simulink model "appendix02_Bicopter_ClosedLoop_PID"  (R2026b)
settings: Solver=FixedStepAuto  StopTime=inf  EnableMultiTasking=on
undefined symbols (not defined in the file or in its folder): ODR
libraries: arduinolib x6, arduinowifilib x2, arduinosensorlib x1, slpidlib x1
settings Model: SILPILModeSetting=veronly  Creator=lcree  LastModifiedBy=ayeo
settings OptimizationCC: DifferentSizesBufferReuse=on  EnhancedBackFolding=on  MaxStackSize=64  OptimizationCustomize=off  OptimizeBlockOrder=speed
settings DebuggingCC: ParameterPrecisionLossMsg=none  ParameterTunabilityLossMsg=error
settings HardwareCC: ProdHWDeviceType=ARM Compatible->ARM Cortex  ProdLargestAtomicFloat=Double  ProdLargestAtomicInteger=Long  UseEmbeddedCoderFeatures=off  UseSimulinkCoderFeatures=off
settings SFSimCC: MATLABDynamicMemAlloc=off
settings RTWCC: BuildConfiguration=Faster Runs  Description=Embedded Coder  HardwareBoard=Arduino Nano 33 IoT  SystemTargetFile=ert.tlc  TLCOptions=-aInlineSetEventsForThisBaseRateFcn=TLC_FALSE -aSuppressMultiTaskScheduler=TLC_FALSE -aRateBasedStepFcn=1  TemplateMakefile=ert_default_tmf  Toolchain=Arduino ARM
settings CodeAppCC: ForceParamTrailComments=on  OperatorAnnotations=on
settings ERTTargetCC: DynamicArrayContainerType=coder::array  ERTCustomFileBanners=off  ExtModeIntrfLevel=Level2 - Open  ExtModeMexFile=ext_xcp  ExtModeStaticAlloc=on  ModelStepFunctionPrototypeControlCompliant=off  SupportContinuousTime=on  SupportNonInlinedSFcns=on  SupportVariableSizeSignals=on

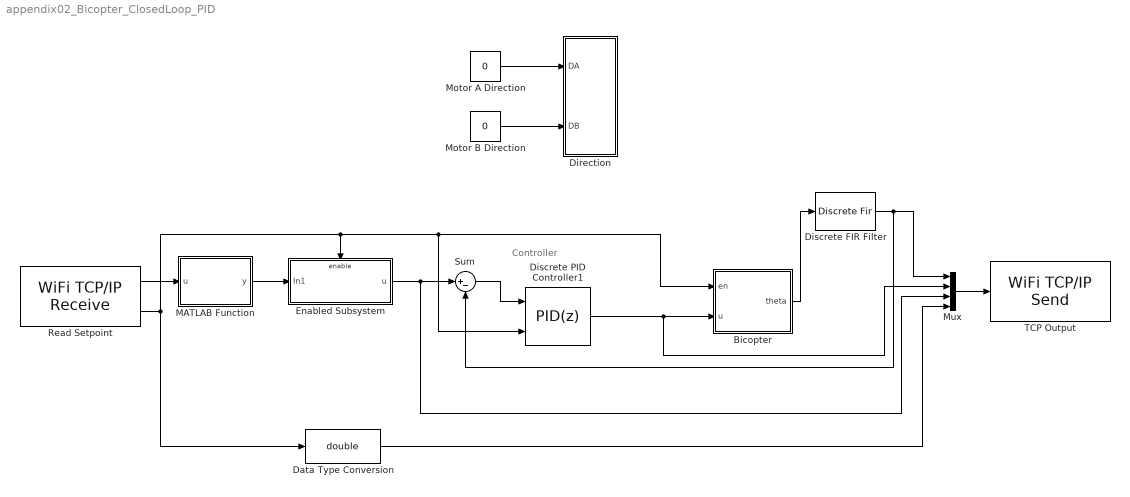
== system appendix02_Bicopter_ClosedLoop_PID ==
  note: Controller
  Bicopter : Subsystem
  Data Type Conversion : DataTypeConversion  OutDataTypeStr=double  SaturateOnIntegerOverflow=off  RndMeth=Floor
  Direction : Subsystem
  Discrete FIR Filter : DiscreteFir  Coefficients=0.1*ones(1,10)  OutDataTypeStr=Inherit: Same as accumulator
  Discrete PID Controller1 : slpidlib/PID Controller  Controller=PID  Form=Parallel  TimeDomain=Discrete-time  UseExternalTs=off  SampleTime=0.01  IntegratorMethod=Backward Euler  FilterMethod=Backward Euler  ControllerParametersSource=internal  P=15.49  I=33.59  UseKiTs=off  D=0  UseExternalDerivativeSource=off  N=100  UseFilter=on  TunerSelectOption=Frequency Response Based  InitialConditionSource=internal  InitialConditionForIntegrator=0  InitialConditionForFilter=0  DifferentiatorICPrevScaledInput=-10  ExternalReset=rising  TrackingMode=off  Kt=1  LimitOutput=off  SatLimitsSource=internal  UpperSaturationLimit=inf  LowerSaturationLimit=-inf  LinearizeAsGain=off  AntiWindupMode=none  Kb=1  LimitIntegrator=off  UpperIntegratorSaturationLimit=inf  LowerIntegratorSaturationLimit=-inf  POutMin=[]  POutMax=[]  IOutMin=[]  IOutMax=[]  DOutMin=[]  DOutMax=[]  NOutMin=[]  NOutMax=[]  SumOutMin=[]  SumOutMax=[]  SaturationOutMin=[]  SaturationOutMax=[]  PParamMin=[]  PParamMax=[]  IParamMin=[]  IParamMax=[]  DParamMin=[]  DParamMax=[]  NParamMin=[]  NParamMax=[]  KbParamMin=[]  KbParamMax=[]  KtParamMin=[]  KtParamMax=[]  KbOutMin=[]  KbOutMax=[]  KtOutMin=[]  KtOutMax=[]  IntegratorOutMin=[]  IntegratorOutMax=[]  FilterOutMin=[]  FilterOutMax=[]  SumI1OutMin=[]  SumI1OutMax=[]  SumI2OutMin=[]  SumI2OutMax=[]  SumI3OutMin=[]  SumI3OutMax=[]  SumI4OutMin=[]  SumI4OutMax=[]  SumDOutMin=[]  SumDOutMax=[]  DifferentiatorOutMin=[]  DifferentiatorOutMax=[]  FilterDiffOutCoefMin=[]  FilterDiffOutCoefMax=[]  ReciprocalOutMin=[]  ReciprocalOutMax=[]  SumDenOutMin=[]  SumDenOutMax=[]  SumNumOutMin=[]  SumNumOutMax=[]  DivideOutMin=[]  DivideOutMax=[]  UdiffTsProdOutMin=[]  UdiffTsProdOutMax=[]  NTsProdOutMin=[]  NTsProdOutMax=[]  UintegralTsProdOutMin=[]  UintegralTsProdOutMax=[]  UngainTsProdOutMin=[]  UngainTsProdOutMax=[]  ClampingZeroOutDataTypeStr=Inherit: Inherit via back propagation  ClampingZeroOutMin=[]  ClampingZeroOutMax=[]  FilterDenConstantOutDataTypeStr=Inherit: Inherit via back propagation  FilterDenConstantOutMin=[]  FilterDenConstantOutMax=[]  PCopyOutDataTypeStr=Inherit: Inherit via back propagation  PCopyOutMin=[]  PCopyOutMax=[]  NCopyOutDataTypeStr=Inherit: Inherit via back propagation  NCopyOutMin=[]  NCopyOutMax=[]  IntegratorContinuousStateAttributes=''  IntegratorStateMustResolveToSignalObject=off  IntegratorRTWStateStorageClass=Auto  FilterContinuousStateAttributes=''  FilterStateMustResolveToSignalObject=off  FilterRTWStateStorageClass=Auto  ParallelPVariant=InternalParameters  IdealPVariant=Disabled  IVariant=InternalParameters  DVariant=InternalParameters  IntegratorVariant=Discrete  SatVariant=Disabled  AWVariant=Passthrough  PCopyVariant=Disabled  TRVariant=Disabled  FdbkBlocksVariant=Forward  IdealPFdbkVariant=Disabled  SatFdbkVariant=Disabled  DerivativeFilterVariant=BackwardEulerFilter  NVariant=InternalParameters  NCopyVariant=InternalParameters  FilterICVariant=InternalICsFilter  IntegratorICVariant=InternalICs  ExternalResetVariant=ExternalReset  TRSumVariant=Passthrough  SumFdbkVariant=Disabled  SumVariant=Sum_PID  TsampFilterVariant=InternalTs  TsampNgainVariant=Passthrough  TsampIntegralVariant=Disabled_SignalSpec  ExternalSaturationOutDataTypeStr=Inherit: Same as second input  DerivativeSourceVariant=ErrorSignal  PreIntVariant=InternalPreInt
  Enabled Subsystem : Subsystem  TreatAsAtomicUnit=on
  MATLAB Function : MATLAB Function  TreatAsAtomicUnit=on
  Motor A Direction : Constant  Value=0  OutDataTypeStr=boolean
  Motor B Direction : Constant  Value=0  OutDataTypeStr=boolean
  Mux : Mux
  Read Setpoint : arduinowifilib/WiFi TCP//IP Receive  Mode_=Server  serverport=25000  RemoteAddr_=192.168.1.2  RemoteServerPort_=25000  DataType_=uint8  DataSize_=4  SampleTime_=0.01  remoteipoctet1=192  remoteipoctet2=168  remoteipoctet3=1  remoteipoctet4=2  wifiTCPServerIndex=0  wifiTCPClientIndex=0  blockPlatform=ARDUINO  isARMArch=true  BlockingMode_=off  BlockTimeout_=1
  Sum : Sum  Inputs=|+-
  TCP Output : arduinowifilib/WiFi TCP//IP Send  Mode_=Server  serverport=25000  RemoteAddr_=192.168.1.2  RemoteServerPort_=25000  remoteipoctet1=192  remoteipoctet2=168  remoteipoctet3=1  remoteipoctet4=2  wifiTCPServerIndex=0  wifiTCPClientIndex=0  blockPlatform=ARDUINO  isARMArch=true
  wires:
  Motor A Direction/1 -> Direction/1(DA)
  Motor B Direction/1 -> Direction/2(DB)
  Mux/1 -> TCP Output/1
  Enabled Subsystem/1(u) -> Sum/1, Mux/3
  Read Setpoint/2 -> Bicopter/1(en), Discrete PID Controller1/2, Enabled Subsystem/Enable, Data Type Conversion/1
  Discrete PID Controller1/1 -> Mux/2, Bicopter/2(u)
  Data Type Conversion/1 -> Mux/4
  Read Setpoint/1 -> MATLAB Function/1(u)
  MATLAB Function/1(y) -> Enabled Subsystem/1(In1)
  Bicopter/1(theta) -> Discrete FIR Filter/1
  Discrete FIR Filter/1 -> Sum/2, Mux/1
  Sum/1 -> Discrete PID Controller1/1

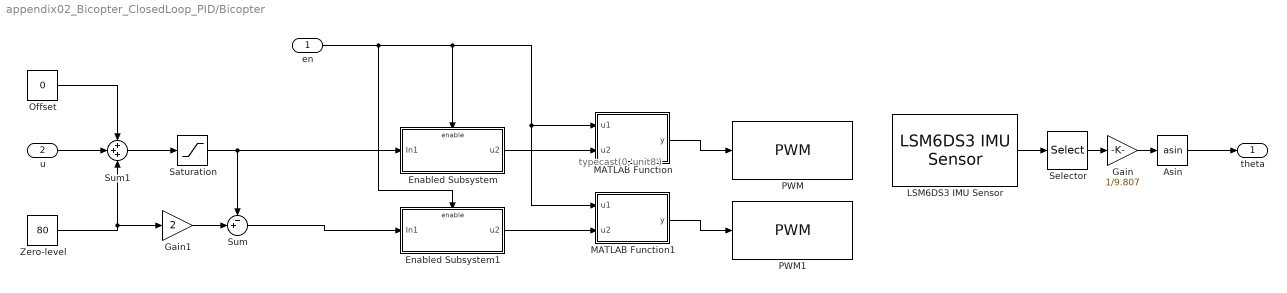
== system appendix02_Bicopter_ClosedLoop_PID/Bicopter ==
  note: typecast(0,'unit8')
  en : Inport
  u : Inport  Port=2
  Asin : Trigonometry  Operator=asin
  Enabled Subsystem : Subsystem  TreatAsAtomicUnit=on
  Enabled Subsystem1 : Subsystem  TreatAsAtomicUnit=on
  Gain : Gain  Gain=1/9.807
  Gain1 : Gain  Gain=2
  LSM6DS3 IMU Sensor : arduinosensorlib/LSM6DS3 IMU Sensor  I2CModule=0  I2CAddress=0x6A  IsActiveAcceleration=on  IsActiveAngularRate=off  IsActiveTemperature=off  IsActiveStatus=off  IsActiveTimeStamp=off  spf=1  SampleTime=0.01  QueueSizeFactor=1  AccelerometerRange=+/- 2g  AccelerometerODR=208 Hz  SelectAnalogBW=off  AccelLPF1BW=400 Hz  AccelSelectCompositeFilter=Low pass filter  AccelLPF2BW=ODR/400  AccelHPFBW=ODR/100  GyroscopeRange=250 dps  GyroscopeODR=12.5 Hz  SelectGyroscopeHPF=off  GyroHPFBW=0.0081 Hz
  MATLAB Function : MATLAB Function  TreatAsAtomicUnit=on
  MATLAB Function1 : MATLAB Function  TreatAsAtomicUnit=on
  Offset : Constant  Value=0
  PWM : arduinolib/PWM  pinNumber=5  frequencyType=Default  desiredFrequency=490.2  achievableFrequency=490.2
  PWM1 : arduinolib/PWM  pinNumber=6  frequencyType=Default  desiredFrequency=490.2  achievableFrequency=490.2
  Saturation : Saturate  UpperLimit=255  LowerLimit=0  OutDataTypeStr=uint8
  Selector : Selector  InputPortWidth=3  IndexOptions=Index vector (dialog)  Indices=[1]  OutputSizes=1  RuntimeRangeChecks=off
  Sum : Sum  Inputs=-+|  OutDataTypeStr=uint8
  Sum1 : Sum  Inputs=+++
  Zero-level : Constant  Value=80
  theta : Outport
  wires:
  LSM6DS3 IMU Sensor/1 -> Selector/1
  Selector/1 -> Gain/1
  Gain1/1 -> Sum/2
  Gain/1 -> Asin/1
  Asin/1 -> theta/1
  Zero-level/1 -> Sum1/3, Gain1/1
  u/1 -> Sum1/2
  Offset/1 -> Sum1/1
  Sum1/1 -> Saturation/1
  en/1 -> Enabled Subsystem/Enable, MATLAB Function1/1(u1), MATLAB Function/1(u1), Enabled Subsystem1/Enable
  Saturation/1 -> Sum/1, Enabled Subsystem/1(In1)
  Sum/1 -> Enabled Subsystem1/1(In1)
  Enabled Subsystem/1(u2) -> MATLAB Function/2(u2)
  MATLAB Function/1(y) -> PWM/1
  Enabled Subsystem1/1(u2) -> MATLAB Function1/2(u2)
  MATLAB Function1/1(y) -> PWM1/1

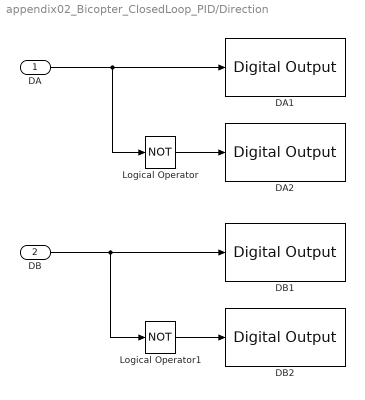
== system appendix02_Bicopter_ClosedLoop_PID/Direction ==
  DA : Inport
  DB : Inport  Port=2
  DA1 : arduinolib/Digital Output  pinNumber=8  Direction=output  blockPlatform=arduino
  DA2 : arduinolib/Digital Output  pinNumber=7  Direction=output  blockPlatform=arduino
  DB1 : arduinolib/Digital Output  pinNumber=3  Direction=output  blockPlatform=arduino
  DB2 : arduinolib/Digital Output  pinNumber=2  Direction=output  blockPlatform=arduino
  Logical Operator : Logic  Operator=NOT  IconShape=distinctive  AllPortsSameDT=off  OutDataTypeStr=boolean
  Logical Operator1 : Logic  Operator=NOT  IconShape=distinctive  AllPortsSameDT=off  OutDataTypeStr=boolean
  wires:
  DB/1 -> Logical Operator1/1, DB1/1
  DA/1 -> Logical Operator/1, DA1/1
  Logical Operator/1 -> DA2/1
  Logical Operator1/1 -> DB2/1

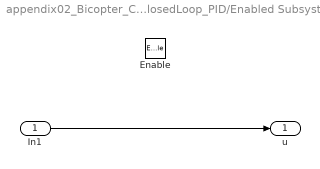
== system appendix02_Bicopter_ClosedLoop_PID/Enabled Subsystem ==
  In1 : Inport
  Enable : EnablePort
  u : Outport
  wires:
  In1/1 -> u/1

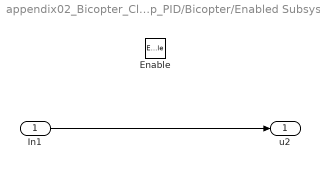
== system appendix02_Bicopter_ClosedLoop_PID/Bicopter/Enabled Subsystem ==
  In1 : Inport
  Enable : EnablePort  StatesWhenEnabling=reset
  u2 : Outport
  wires:
  In1/1 -> u2/1

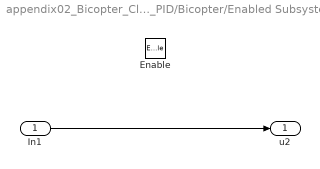
== system appendix02_Bicopter_ClosedLoop_PID/Bicopter/Enabled Subsystem1 ==
  In1 : Inport
  Enable : EnablePort  StatesWhenEnabling=reset
  u2 : Outport
  wires:
  In1/1 -> u2/1

== matlab function appendix02_Bicopter_ClosedLoop_PID/MATLAB Function ==
  data: u input uint8 size=4; y output double size=1
function y = fcn(u)
y = double(typecast(u,'single'));
end

== matlab function appendix02_Bicopter_ClosedLoop_PID/Bicopter/MATLAB Function1 ==
  data: u1 input; y output; u2 input
function y  = fcn(u1,u2)
y=uint8(0);
if u1 == 1
    y=uint8(u2);
end

== matlab function appendix02_Bicopter_ClosedLoop_PID/Bicopter/MATLAB Function ==
  data: u1 input; y output; u2 input
function y  = fcn(u1,u2)
y=uint8(0);
if u1 == 1
    y=uint8(u2);
end
